simulink model "test_v2"  (Simulink 7.0)
settings: Solver=FixedStepDiscrete  StartTime=0.0  StopTime=inf  FixedStep=0.01  RelTol=1e-3
libraries: xpcutilitieslib x11, dsPICdrivers x7
settings Model: Creator=sathish  LastModifiedBy=sathish  TunableVars=ONE,ZERO  TunableVarsStorageClass=ExportedGlobal,ExportedGlobal  TunableVarsTypeQualifier=const,const
settings DataIOCC: LimitDataPoints=off  SaveOutput=off  SignalLogging=off  SaveTime=off
settings OptimizationCC: InlineParams=on  OptimizeModelRefInitCode=on  LifeSpan=1
settings DebuggingCC: SaveWithParameterizedLinksMsg=none
settings HardwareCC: ProdBitPerInt=16  ProdEndianess=LittleEndian  ProdWordSize=16  ProdHWDeviceType=16-bit Generic  TargetHWDeviceType=32-bit Generic
settings RTWCC: SystemTargetFile=dspic.tlc  GenCodeOnly=on  TemplateMakefile=dspic_pic30_gcc.tmf  PostCodeGenCommand=dsPIC_Compile()  Description=Embedded Target for Microchip dsPIC (real-time)  ProcessScript=dspic_make_rtw_hook  CustomSourceCode="#include \"C:\\Program Files\\Microchip\\MPLAB C30\\src\\peripheral_30F_24H_33F\\src\\pmc\\timer\\ConfigIntTimer1.c\""  CustomInclude=C:\Users\sathish\Desktop\temp\ou(2)\lib
settings CodeAppCC: IgnoreCustomStorageClasses=off
settings STFCustomTargetCC: GenFloatMathFcnCalls=ANSI_C  ModelReferenceCompliant=off  IncludeMdlTerminateFcn=off  CombineOutputUpdateFcns=on  SuppressErrorStatus=on  ERTCustomFileBanners=on  SupportContinuousTime=off  SupportNonInlinedSFcns=off  SystemTargetFile=dspic.tlc
settings ERTTargetCC: GenFloatMathFcnCalls=ANSI_C  ModelReferenceCompliant=off  CompOptLevelCompliant=off  IncludeMdlTerminateFcn=off  SuppressErrorStatus=on  ModelStepFunctionPrototypeControlCompliant=off  ExtModeMexFile=noextcomm  InlinedParameterPlacement=NonHierarchical  ERTSrcFileBannerTemplate=dsPIC_code_template.cgt  ERTHdrFileBannerTemplate=dsPIC_code_template.cgt  ERTDataSrcFileTemplate=dsPIC_code_template.cgt  ERTDataHdrFileTemplate=dsPIC_code_template.cgt  ERTCustomFileTemplate=dsPIC_main.tlc
settings CustomProperty: DataType=string  Value=C:\MAD7D5~1\bin\win32\gmake

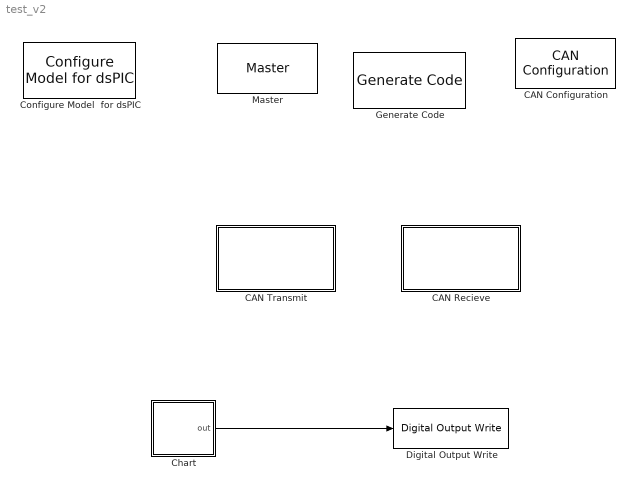
== system test_v2 ==
  CAN Configuration : dsPICdrivers/BUS CAN/CAN Configuration  Tag=dsPIC_CAN_Config  NumCAN=1  Mode=Normal  TcanTcy="Tcan  = Tcy/4"  BRP=0  PRSEG=1  SEG1PH=4  SAM_popup=Once at sample point  SEG2PH=1  SJW=1  SampleTime=-1  OrderingInOutPopup=None  Info="Tq = 5e-007s   X 8  -->  Fcan = 250 KHz"
  CAN Recieve : Subsystem  TreatAsAtomicUnit=on
  CAN Transmit : Subsystem  TreatAsAtomicUnit=on
  Chart : Stateflow chart
  Configure Model  for dsPIC : dsPICdrivers/Simulink Configuration/Configure Model  for dsPIC
  Digital Output Write : dsPICdrivers/Digital I//O/Digital Output Write  Tag=dsPIC_Digital_Output  Priority=5  PORT=B  Pin=[0]  Simultaneous=off  OrderingInOutPopup=None
  Generate Code : dsPICdrivers/Simulink Configuration/Generate Code
  Master : dsPICdrivers/Master  Tag=dsPIC_MASTER  Priority=1  TimeStepType=Timer1  picType=30f4011  fcy=16e6  Quartz_33f=5e6  PLLActive_33f=off  fcyDesired_33f=0  tmr1="[1  9999  0]"  tmr1Info="Time Step : 0.01  ;   Error : 0%  PR1=9999"  tmr2345="[0  0  0  0]"  tmr2345cfg=[-1 -1 -1 -1]  IOautoConf=on  typePort="[ 0   0   0   0   0   0   0   0   0   0   0   0   0   0   0   0  10   0   0   0   0   0   0   0   0   0   0   0   0   0   0   0   0   0   0   0   0   0   0   0   0   0   0   0   0   0   0   0   0   0   0   0   0   0   0   0   0   0   0   0   0   0   0   0   0   0   0   0   0   0   0   0   0   0   0   0   0   0   0   0  19  19   0   0   0   0   0   0   0   0   0   0   0   0   0   0   0   0   0   0   0   0   0   0   0   0   0   0   0   0   0   0 ]"  TRIS="[ 65535  65534  65535  65535  65535  65535  65535 ]"  ADPCFG=1  MasterBusyPort=None  MasterOverloadPort=None  FOSC=XT_PLL8  ClockSwitchMonitor=Both disabled  TempProtection_33f=TEMP_ON  FPBOR=PBOR_OFF  PWRT=PWRT_OFF  MCLR=MCLR_EN  PowerSave=off  OverrideFcy=on  NewFcy=1e6  PR2345="[65535  65535  65535  65535]"
  wires:
  Chart/1(out) -> Digital Output Write/1

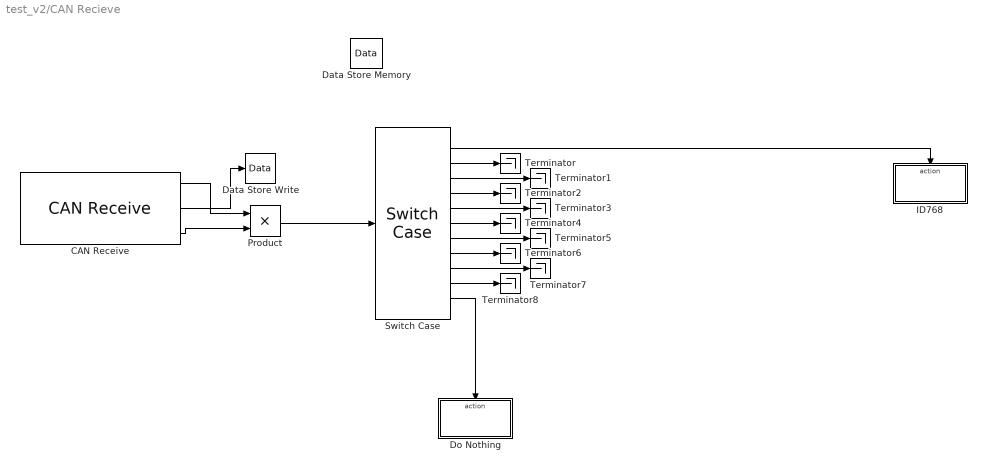
== system test_v2/CAN Recieve ==
  CAN Receive : dsPICdrivers/BUS CAN/CAN Receive  Tag=dsPIC_CAN_Receive  NumCAN=1  RXM0=777  DL0=8  RXF0=0  F0type=Standard or Extended  DL0received=off  FlagNewMessage0=on  OutId0=on  DataRequestSend0=off  DL1=Off  RXF1=0  F1type=Standard or Extended  DL1received=off  FlagNewMessage1=off  OutId1=off  DataRequestSend1=off  RXM1=0  DL2=Off  RXF2=0  F2type=Standard or Extended  DL2received=off  FlagNewMessage2=off  OutId2=off  DataRequestSend2=off  DL3=Off  RXF3=0  F3type=Standard or Extended  DL3received=off  FlagNewMessage3=off  OutId3=off  DataRequestSend3=off  DL4=Off  RXF4=0  F4type=Standard or Extended  DL4received=off  FlagNewMessage4=off  OutId4=off  DataRequestSend4=off  DBEN=off  ErrCount=off  DataLost=off  SampleTime=-1  OrderingInOutPopup=None  Info=0
  Data Store Memory : DataStoreMemory  DataStoreName=Data  ReadBeforeWriteMsg=warning  WriteAfterWriteMsg=warning  WriteAfterReadMsg=warning  InitialValue=[0 0 0 0 0 0 0 0]  OutDataType=sfix(16)  OutScaling=2^0
  Data Store Write : DataStoreWrite  DataStoreName=Data  SampleTime=-1
  Do Nothing : Subsystem  TreatAsAtomicUnit=on
  ID768 : Subsystem  TreatAsAtomicUnit=on
  Product : Product  OutDataType=sfix(16)  OutScaling=2^0  RndMeth=Zero
  Switch Case : SwitchCase  CaseConditions={768 769 770 771 772 773 774 775 776 777}
  Terminator{,1..8} (9 alike) : Terminator
  wires:
  Switch Case/11 -> Do Nothing/Action
  Switch Case/1 -> ID768/Action
  CAN Receive/3 -> Product/2
  Product/1 -> Switch Case/1
  CAN Receive/1 -> Product/1
  CAN Receive/2 -> Data Store Write/1
  Switch Case/2 -> Terminator/1
  Switch Case/3 -> Terminator1/1
  Switch Case/4 -> Terminator2/1
  Switch Case/5 -> Terminator3/1
  Switch Case/6 -> Terminator4/1
  Switch Case/7 -> Terminator5/1
  Switch Case/8 -> Terminator6/1
  Switch Case/9 -> Terminator7/1
  Switch Case/10 -> Terminator8/1

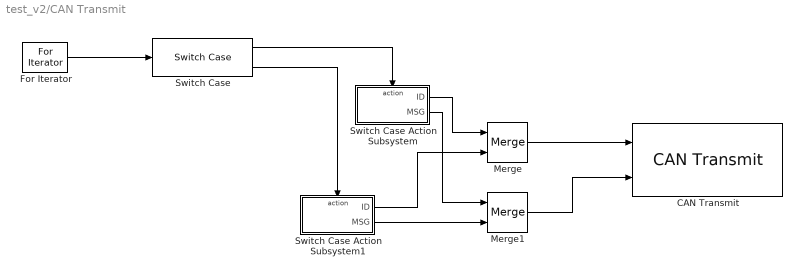
== system test_v2/CAN Transmit ==
  CAN Transmit : dsPICdrivers/BUS CAN/CAN Transmit  Tag=dsPIC_CAN_Transmit  NumCAN=1  WaitPreviousTransmission=off  TxPriority=Highest  IdentifierType=Standard 11 bits  IdentifierBlockInput=on  Identifier=[256]  SRR=Normal Message  DLC=8  TransmitBlockInput=on  TransmitValue=0  TxFull=off  OutErrCount=off  TXBO=off  TXEP=off  TXWAR=off  SampleTime=-1  OrderingInOutPopup=None  Info=0
  For Iterator : ForIterator  IterationLimit=2  IterationVariableDataType=int8
  Merge : Merge
  Merge1 : Merge  InitialOutput=[0 0 0 0 0 0 0 0]
  Switch Case : SwitchCase
  Switch Case Action Subsystem : Subsystem  TreatAsAtomicUnit=on
  Switch Case Action Subsystem1 : Subsystem  TreatAsAtomicUnit=on
  wires:
  For Iterator/1 -> Switch Case/1
  Switch Case/1 -> Switch Case Action Subsystem/Action
  Switch Case/2 -> Switch Case Action Subsystem1/Action
  Switch Case Action Subsystem/1(ID) -> Merge/1
  Switch Case Action Subsystem1/1(ID) -> Merge/2
  Merge/1 -> CAN Transmit/1
  Switch Case Action Subsystem/2(MSG) -> Merge1/1
  Switch Case Action Subsystem1/2(MSG) -> Merge1/2
  Merge1/1 -> CAN Transmit/2

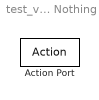
== system test_v2/CAN Recieve/Do Nothing ==
  Action Port : ActionPort  ActionType=default

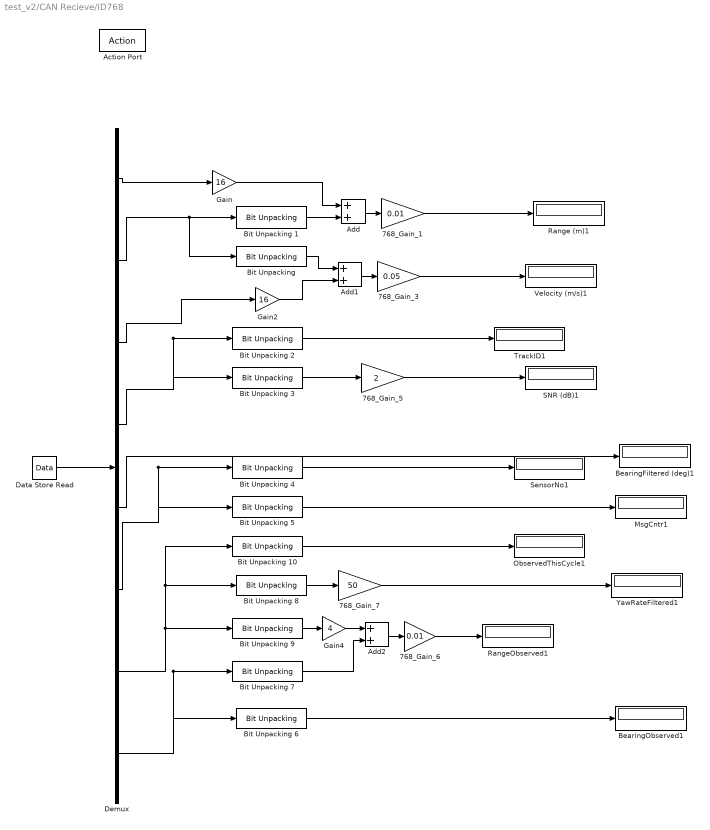
== system test_v2/CAN Recieve/ID768 ==
  Action Port : ActionPort  ActionType=case
  768_Gain_1 : Gain  Gain=0.01  ParameterDataType=sfix(16)  ParameterScaling=2^0  OutDataType=sfix(16)  OutScaling=2^0
  768_Gain_3 : Gain  Gain=0.05  ParameterDataType=sfix(16)  ParameterScaling=2^0  OutDataType=sfix(16)  OutScaling=2^0
  768_Gain_5 : Gain  Gain=2  ParameterDataType=sfix(16)  ParameterScaling=2^0  OutDataType=sfix(16)  OutScaling=2^0
  768_Gain_6 : Gain  Gain=0.01  ParameterDataType=sfix(16)  ParameterScaling=2^0  OutDataType=sfix(16)  OutScaling=2^0
  768_Gain_7 : Gain  Gain=50  ParameterDataType=sfix(16)  ParameterScaling=2^0  OutDataType=sfix(16)  OutScaling=2^0
  Add : Sum  OutDataType=sfix(16)  OutScaling=2^-10
  Add1 : Sum  OutDataType=sfix(16)  OutScaling=2^-10
  Add2 : Sum  OutDataType=sfix(16)  OutScaling=2^-10
  BearingFiltered (deg)1 : Display
  BearingObserved1 : Display
  Bit Unpacking {,1..10} (11 alike) : xpcutilitieslib/Bit Unpacking   SignExtend=on
  Data Store Read : DataStoreRead  DataStoreName=Data  SampleTime=-1
  Demux : Demux  Outputs=8
  Gain : Gain  Gain=16  ParameterDataType=sfix(16)  ParameterScaling=2^0  OutDataType=sfix(16)  OutScaling=2^0
  Gain2 : Gain  Gain=16  ParameterDataType=sfix(16)  ParameterScaling=2^0  OutDataType=sfix(16)  OutScaling=2^0
  Gain4 : Gain  Gain=4  ParameterDataType=sfix(16)  ParameterScaling=2^0  OutDataType=sfix(16)  OutScaling=2^0
  MsgCntr1 : Display
  ObservedThisCycle1 : Display
  Range (m)1 : Display
  RangeObserved1 : Display
  SNR (dB)1 : Display
  SensorNo1 : Display
  TrackID1 : Display
  Velocity (m/s)1 : Display
  YawRateFiltered1 : Display
  wires:
  Demux/1 -> Gain/1
  Demux/2 -> "Bit Unpacking "/1, Bit Unpacking 1/1
  Bit Unpacking 1/1 -> Add/2
  Gain/1 -> Add/1
  Add/1 -> 768_Gain_1/1
  Demux/3 -> Gain2/1
  Add1/1 -> 768_Gain_3/1
  "Bit Unpacking "/1 -> Add1/1
  Gain2/1 -> Add1/2
  Demux/4 -> Bit Unpacking 2/1, Bit Unpacking 3/1
  Bit Unpacking 3/1 -> 768_Gain_5/1
  Demux/6 -> Bit Unpacking 4/1, Bit Unpacking 5/1
  Bit Unpacking 8/1 -> 768_Gain_7/1
  Demux/8 -> Bit Unpacking 7/1, Bit Unpacking 6/1
  Bit Unpacking 9/1 -> Gain4/1
  Gain4/1 -> Add2/1
  Bit Unpacking 7/1 -> Add2/2
  Add2/1 -> 768_Gain_6/1
  768_Gain_1/1 -> Range (m)1/1
  768_Gain_3/1 -> Velocity (m/s)1/1
  Bit Unpacking 2/1 -> TrackID1/1
  768_Gain_5/1 -> SNR (dB)1/1
  Demux/5 -> BearingFiltered (deg)1/1
  Bit Unpacking 4/1 -> SensorNo1/1
  Bit Unpacking 5/1 -> MsgCntr1/1
  Bit Unpacking 10/1 -> ObservedThisCycle1/1
  768_Gain_7/1 -> YawRateFiltered1/1
  768_Gain_6/1 -> RangeObserved1/1
  Bit Unpacking 6/1 -> BearingObserved1/1
  Demux/7 -> Bit Unpacking 9/1, Bit Unpacking 8/1, Bit Unpacking 10/1
  Data Store Read/1 -> Demux/1

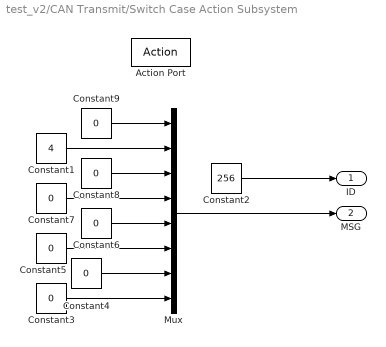
== system test_v2/CAN Transmit/Switch Case Action Subsystem ==
  Action Port : ActionPort  ActionType=case
  Constant1 : Constant  Value=4  OutDataTypeMode=uint8  OutDataType=sfix(16)  OutScaling=2^0  SampleTime=-1
  Constant2 : Constant  Value=256  OutDataTypeMode=uint16  OutDataType=sfix(16)  OutScaling=2^0  SampleTime=-1
  Constant{3..9} (7 alike) : Constant  Value=0  OutDataTypeMode=uint8  OutDataType=sfix(16)  OutScaling=2^0  SampleTime=-1
  Mux : Mux  Inputs=8
  ID : Outport  OutDataType=sfix(16)  OutScaling=2^0
  MSG : Outport  Port=2  OutDataType=sfix(16)  OutScaling=2^0
  wires:
  Constant1/1 -> Mux/2
  Constant2/1 -> ID/1
  Mux/1 -> MSG/1
  Constant7/1 -> Mux/4
  Constant8/1 -> Mux/3
  Constant6/1 -> Mux/5
  Constant5/1 -> Mux/6
  Constant4/1 -> Mux/7
  Constant3/1 -> Mux/8
  Constant9/1 -> Mux/1

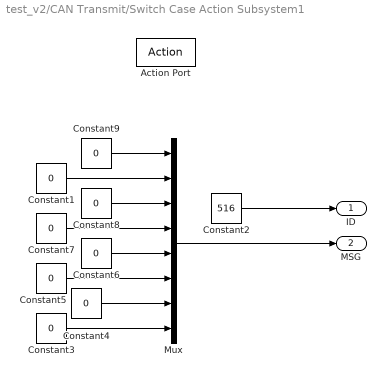
== system test_v2/CAN Transmit/Switch Case Action Subsystem1 ==
  Action Port : ActionPort  ActionType=default
  Constant{1,3..9} (8 alike) : Constant  Value=0  OutDataTypeMode=uint8  OutDataType=sfix(16)  OutScaling=2^0  SampleTime=-1
  Constant2 : Constant  Value=516  OutDataTypeMode=uint16  OutDataType=sfix(16)  OutScaling=2^0
  Mux : Mux  Inputs=8
  ID : Outport  OutDataType=sfix(16)  OutScaling=2^0
  MSG : Outport  Port=2  OutDataType=sfix(16)  OutScaling=2^0
  wires:
  Constant2/1 -> ID/1
  Mux/1 -> MSG/1
  Constant1/1 -> Mux/2
  Constant7/1 -> Mux/4
  Constant8/1 -> Mux/3
  Constant6/1 -> Mux/5
  Constant5/1 -> Mux/6
  Constant4/1 -> Mux/7
  Constant3/1 -> Mux/8
  Constant9/1 -> Mux/1

== stateflow chart Chart ==
  state ON/
    en: out = TRUE;
    time = 0;
    du: time = time + 0.01;
  state OFF/
    en: out = FALSE;
    time = 0;
    du: time = time + 0.01;
  ON -> OFF : [time >= 0.02]
  OFF -> ON : [time >= 0.02]
  (default) -> ON
  data: out output boolean; FALSE constant boolean =0; TRUE constant boolean =1; time local double
